simulink model "SensorlessFOC"  (R2026b)
settings: Solver=ode4  StopTime=experimentCfg.Duration  FixedStep=experimentCfg.Step
PostLoadFcn:
  | addpath(fullfile(fileparts(get_param(bdroot,'FileName')),'..','build_process'));initialize_sensorless_foc(bdroot);
model workspace (MAT data in the model file):
  currentCfg.Ts = 5e-05
  currentCfg.BandwidthHz = 500
  currentCfg.Kpd = 3.14159265359
  currentCfg.Kpq = 3.14159265359
  currentCfg.Kid = 1570.79632679
  currentCfg.Kiq = 1570.79632679
  currentCfg.Kaw = 20000
  deadtimeCfg.DeadTime = 2e-06
  deadtimeCfg.DeviceDrop = 0
  deadtimeCfg.CurrentBlend = 0.1
  deadtimeCfg.ModelEnable = 0
  deadtimeCfg.CompensationEnable = 0
  deadtimeCfg.CompensationScale = 1
  deadtimeCfg.SwitchingStep = 1e-07
  experimentCfg.UseInverter = 1
  experimentCfg.UseTiming = 1
  experimentCfg.Step = 5e-06
  experimentCfg.LogTs = 5e-05
  experimentCfg.Duration = 2
  focCfg.Direction = 1
  focCfg.SpeedReference = 80
  focCfg.SpeedInitial = 0
  focCfg.CommandTime = 0.05
  focCfg.LoadTorque = 0.1
  focCfg.LoadTime = 0.9
  focCfg.Enable = 1
  focCfg.Reset = 0
  focCfg.ObserverEnable = 1
  focCfg.CurrentMax = 8
  focCfg.Kt = 0.21
  focCfg.VoltageAlignmentEnable = 1
  focCfg.AlignmentVoltageGain = 0.5
  focCfg.FrameCorrectionTolerance = 1e-10
  handoverCfg.Ts = 5e-05
  handoverCfg.MinOmega = 100
  handoverCfg.MaxSpeedGap = 80
  handoverCfg.MaxPhaseGap = 0.9
  handoverCfg.MaxResidual = 1.5
  handoverCfg.CaptureTime = 0.01
  handoverCfg.BlendTime = 0.1
  handoverCfg.LossTime = 0.001
  handoverCfg.MaxPhaseInnovation = 0.15
  handoverCfg.AllowFlying = 0
  handoverCfg.Samples = [200; 2000; 20]
  handoverCfg.Vector = [5e-05; 100; 80; 0.9; 1.5; 200; 2000; 20; 0.15; 0]
  handoverCfg.State0 = [0; 0; 0; 0; 0; 0; 0; 0; 0]
  inverterCfg.Vdc = 48
  inverterCfg.MinDuty = 0.02
  inverterCfg.PwmTs = 5e-05
  inverterCfg.LinearLimit = 26.6043004043
  motionCfg.Ts = 0.001
  motionCfg.NaturalFrequency = 20
  motionCfg.Damping = 0.9
  motionCfg.Kt = 0.21
  motionCfg.Kp = 0.0852380952381
  motionCfg.Ki = 0.952380952381
  motionCfg.Kaw = 20
  motionCfg.PositionKp = 8
  motionCfg.SpeedLimit = 120
  motionCfg.AccelerationLimit = 200
  motionCfg.CurrentLimit = 8
  pllCfg.Ts = 5e-05
  pllCfg.NaturalFrequency = 40
  pllCfg.Damping = 0.707
  pllCfg.Kp = 355.376960974
  pllCfg.Ki = 63165.468167
  pllCfg.Kaw = 502.654824574
  pllCfg.OmegaMax = 1500
  pllCfg.MinMagnitude = 1
  pllCfg.LockError = 0.12
  pllCfg.LockSamples = 100
  pllCfg.Theta0 = 0
  pllCfg.Omega0 = 0
  pmsmCfg.Rs = 0.5
  pmsmCfg.Ld = 0.001
  pmsmCfg.Lq = 0.001
  pmsmCfg.Flux = 0.035
  pmsmCfg.PolePairs = 4
  pmsmCfg.J = 0.0005
  pmsmCfg.B = 0.0001
  pmsmCfg.Id0 = 0
  pmsmCfg.Iq0 = 0
  pmsmCfg.Speed0 = 0
  pmsmCfg.Position0 = 0.1
  refCfg.SpeedTs = 0.001
  refCfg.SpeedKp = 0.0179
  refCfg.SpeedKi = 0.2
  refCfg.SpeedKaw = 1000
  smoCfg.Ts = 5e-05
  smoCfg.Rs = 0.5
  smoCfg.L = 0.001
  smoCfg.Flux = 0.035
  smoCfg.PolePairs = 4
  smoCfg.SlidingGain = 30
  smoCfg.Boundary = 1
  smoCfg.FilterHz = 600
  smoCfg.MinEmf = 1
  smoCfg.MinOmega = 30
  smoCfg.Compensate = 1
  smoCfg.A = 0.975309912028
  smoCfg.B = 0.0493801759433
  smoCfg.FilterA = 0.828204181307
  smoCfg.BoundaryPole = -0.506095366272
  startupCfg.Ts = 5e-05
  startupCfg.Theta0 = 0
  startupCfg.AlignCurrent = 2
  startupCfg.StartupCurrent = 3
  startupCfg.FinalOmega = 250
  startupCfg.FlyingCaptureTime = 0.03
  startupCfg.PrealignTime = 0.06
  startupCfg.PrealignRampTime = 0.03
  startupCfg.AlignTime = 0.08
  startupCfg.AlignRampTime = 0.04
  startupCfg.OmegaRampTime = 0.35
  startupCfg.CurrentRampTime = 0.05
  startupCfg.MinCaptureOmega = 150
  startupCfg.MaxIFTime = 0.8
  startupCfg.Samples = [600 1200 600 1600 800 7000 1000 16000]
  startupCfg.Vector = [5e-05; 0; 2; 3; 250; 600; 1200; 600; 1600; 800; 7000; 1000; 16000; 150]
  startupCfg.State0 = [0; 0; 0; 0; 0]
  testStim.time = [0 5e-05 0.0001 0.00015 0.0002 0.00025 0.0003 0.00035 0.0004 0.00045 0.0005 0.00055 ... (40001 elements, 40001x1)]
  testStim.signals.values = [0 0 0 0 0 0 0 0 0 0 0 0 ... (240006 elements, 40001x6)]
  testStim.signals.dimensions = 6
  timingCfg.Ts = 5e-05
  timingCfg.FeedbackTicks = 0
  timingCfg.ActuationTicks = 1
libraries: ClarkePark x14, Inverter x3, CurrentControl x2, PMSMPlant x2, Deadtime x2, SensorlessHandover x1, CurrentReference x1, SensorlessStartup x1, SlidingModeObserver x1, ControlTiming x1
settings Model: Creator=24322  LastModifiedBy=24322

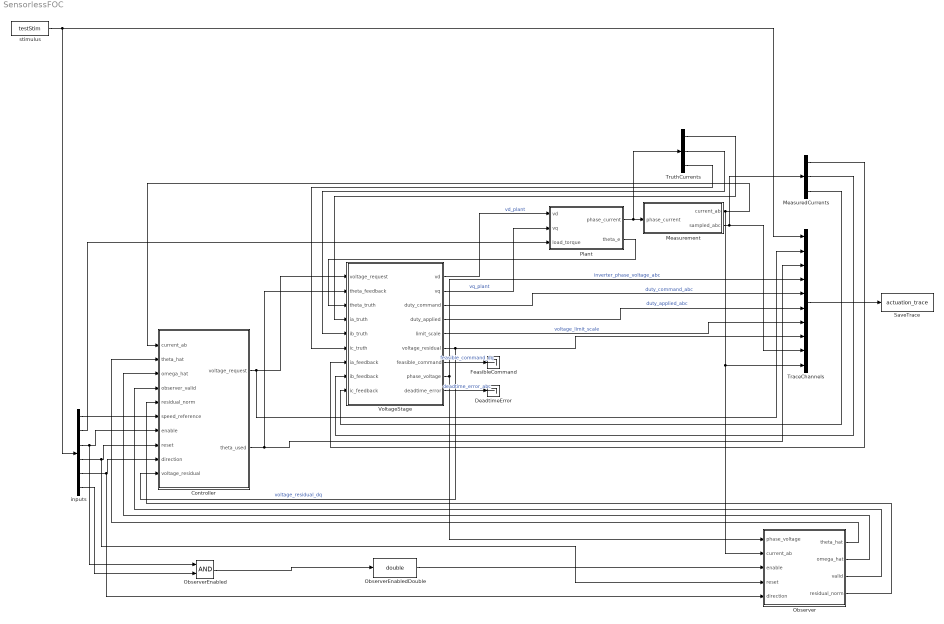
== system SensorlessFOC ==
  Controller : Subsystem
  DeadtimeError : Terminator
  FeasibleCommand : Terminator
  MeasuredCurrents : Demux  Outputs=3
  Measurement : Subsystem
  Observer : Subsystem
  ObserverEnabled : Logic  IconShape=distinctive  AllPortsSameDT=off  OutDataTypeStr=boolean
  ObserverEnabledDouble : DataTypeConversion  OutDataTypeStr=double  SaturateOnIntegerOverflow=off  RndMeth=Floor
  Plant : Subsystem
  SaveTrace : ToWorkspace  VariableName=actuation_trace  SaveFormat=Structure With Time  SampleTime=currentCfg.Ts
  TraceChannels : Mux  Inputs=10
  TruthCurrents : Demux  Outputs=3
  VoltageStage : Subsystem
  inputs : Demux  Outputs=6
  stimulus : FromWorkspace  VariableName=testStim  SampleTime=currentCfg.Ts  Interpolate=off  OutputAfterFinalValue=Holding final value
  wires:
  VoltageStage/5(limit_scale) -> TraceChannels/7  "voltage_limit_scale"
  VoltageStage/4(duty_applied) -> TraceChannels/6  "duty_applied_abc"
  VoltageStage/3(duty_command) -> TraceChannels/5  "duty_command_abc"
  TraceChannels/1 -> SaveTrace/1
  MeasuredCurrents/3 -> VoltageStage/9(ic_feedback)
  TruthCurrents/3 -> VoltageStage/6(ic_truth)
  MeasuredCurrents/2 -> VoltageStage/8(ib_feedback)
  TruthCurrents/2 -> VoltageStage/5(ib_truth)
  MeasuredCurrents/1 -> VoltageStage/7(ia_feedback)
  TruthCurrents/1 -> VoltageStage/4(ia_truth)
  VoltageStage/9(deadtime_error) -> DeadtimeError/1  "deadtime_error_abc"
  VoltageStage/7(feasible_command) -> FeasibleCommand/1  "feasible_command_dq"
  VoltageStage/6(voltage_residual) -> Controller/10(voltage_residual), TraceChannels/8  "voltage_residual_dq"
  inputs/1 -> Controller/6(speed_reference)
  Observer/4(residual_norm) -> Controller/5(residual_norm)
  Observer/3(valid) -> Controller/4(observer_valid)
  Observer/2(omega_hat) -> Controller/3(omega_hat)
  Observer/1(theta_hat) -> Controller/2(theta_hat)
  inputs/5 -> Observer/5(direction), Controller/9(direction)
  inputs/4 -> Observer/4(reset), Controller/8(reset)
  ObserverEnabledDouble/1 -> Observer/3(enable)
  Measurement/1(current_ab) -> TraceChannels/10, Observer/2(current_ab), Controller/1(current_ab)
  VoltageStage/8(phase_voltage) -> Observer/1(phase_voltage), TraceChannels/4  "inverter_phase_voltage_abc"
  Measurement/2(sampled_abc) -> MeasuredCurrents/1, TraceChannels/9
  Plant/1(phase_current) -> Measurement/1(phase_current), TruthCurrents/1
  inputs/2 -> Plant/3(load_torque)
  VoltageStage/2(vq) -> Plant/2(vq)  "vq_plant"
  VoltageStage/1(vd) -> Plant/1(vd)  "vd_plant"
  Plant/2(theta_e) -> VoltageStage/3(theta_truth)
  Controller/2(theta_used) -> VoltageStage/2(theta_feedback), TraceChannels/3
  Controller/1(voltage_request) -> VoltageStage/1(voltage_request), TraceChannels/2
  ObserverEnabled/1 -> ObserverEnabledDouble/1
  inputs/6 -> ObserverEnabled/2
  inputs/3 -> ObserverEnabled/1, Controller/7(enable)
  stimulus/1 -> inputs/1, TraceChannels/1

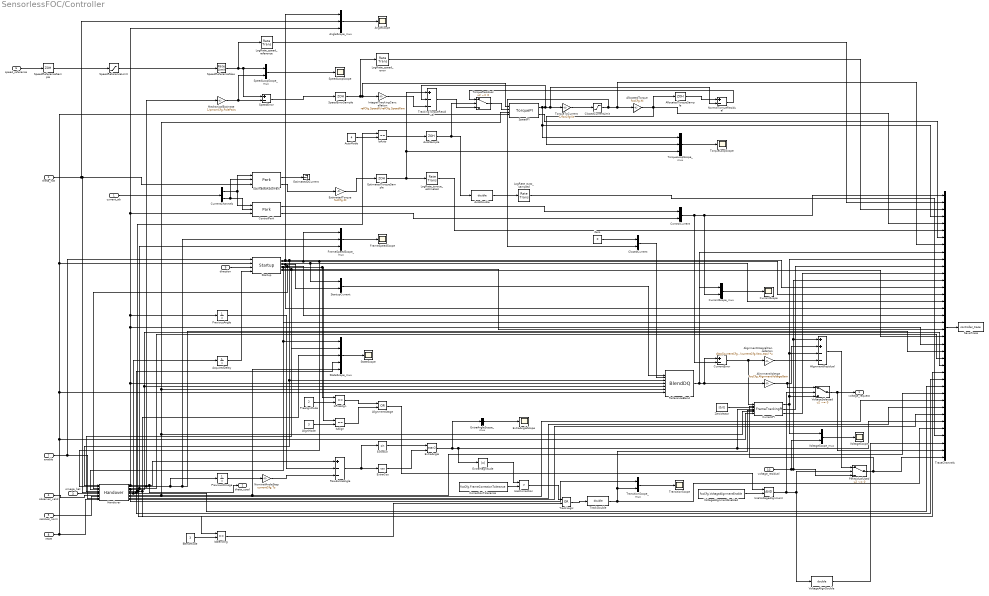
== system SensorlessFOC/Controller ==
  current_ab : Inport
  theta_hat : Inport  Port=2
  omega_hat : Inport  Port=3
  observer_valid : Inport  Port=4
  residual_norm : Inport  Port=5
  speed_reference : Inport  Port=6
  enable : Inport  Port=7
  reset : Inport  Port=8
  direction : Inport  Port=9
  voltage_residual : Inport  Port=10
  AcquiredDelay : UnitDelay  SampleTime=currentCfg.Ts
  AlignMode : Constant  Value=3
  AlignmentIntegralCancellation : Gain  Gain=diag([currentCfg.Kid,currentCfg.Kiq])/max(currentCfg.Kaw,eps)  Multiplication=Matrix(K*u)
  AlignmentResidual : Sum  Inputs=++--
  AlignmentStage : Logic  Operator=OR  IconShape=distinctive  AllPortsSameDT=off  OutDataTypeStr=boolean
  AlignmentVoltage : Gain  Gain=focCfg.AlignmentVoltageGain
  AllocatedTorque : Gain  Gain=focCfg.Kt
  AllocatedTorqueSample : ZeroOrderHold  SampleTime=refCfg.SpeedTs
  AngleScope : Scope
  AngleScope_mux : Mux  Inputs=3
  AutoDouble : DataTypeConversion  OutDataTypeStr=double  SaturateOnIntegerOverflow=off  RndMeth=Floor
  AutoMode : Constant  Value=4
  AutoSample : ZeroOrderHold  SampleTime=refCfg.SpeedTs
  BlendMode : Constant  Value=3
  ClosedCurrent : Mux  Inputs=2
  ClosedCurrentLimit : Saturate  UpperLimit=focCfg.CurrentMax  LowerLimit=-focCfg.CurrentMax
  ControlCurrent : Mux  Inputs=2
  ControlPark : ClarkePark/Park  SystemSampleTime=-1  VariantActivationTime=update diagram  EmptyChoice=off  PassThrough=off  PassThroughVariantControl=(default)  EmptyChoiceVariantControl=(default)  AllowFlexibleInterface=on  Latency=0  AutoFrameSizeCalculation=off
  CorrectionTolerance : Constant  Value=focCfg.FrameCorrectionTolerance
  CurrentChannels : Demux  Outputs=2
  CurrentError : Sum  Inputs=+-
  CurrentPI : CurrentControl/FrameTrackingPI  currentCfg=currentCfg
  CurrentScope : Scope
  CurrentScope_mux : Mux  Inputs=2
  EstimatedDCurrent : Terminator
  EstimatedRotorPark : ClarkePark/Park  SystemSampleTime=-1  VariantActivationTime=update diagram  EmptyChoice=off  PassThrough=off  PassThroughVariantControl=(default)  EmptyChoiceVariantControl=(default)  AllowFlexibleInterface=on  Latency=0  AutoFrameSizeCalculation=off
  EstimatedTorque : Gain  Gain=focCfg.Kt
  EstimatedTorqueSample : ZeroOrderHold  SampleTime=refCfg.SpeedTs
  ExtraAngle : Trigonometry  Operator=atan2
  ExtraAngleScope : Scope
  ExtraAngleScope_mux : Mux  Inputs=1
  ExtraCos : Trigonometry  Operator=cos
  ExtraMagnitude : Abs  SaturateOnIntegerOverflow=off
  ExtraSin : Trigonometry
  FrameSpeedScope : Scope
  FrameSpeedScope_mux : Mux  Inputs=3
  Handover : SensorlessHandover/Handover  handoverCfg=handoverCfg
  HasCorrection : RelationalOperator  Operator=>  OutDataTypeStr=boolean  RndMeth=Simplest  InputSameDT=off
  IntegralTrackingCancellation : Gain  Gain=refCfg.SpeedKi/refCfg.SpeedKaw
  IsAlign : RelationalOperator  Operator===  OutDataTypeStr=boolean  RndMeth=Simplest  InputSameDT=off
  IsAuto : RelationalOperator  Operator===  OutDataTypeStr=boolean  RndMeth=Simplest  InputSameDT=off
  IsBlending : RelationalOperator  Operator===  OutDataTypeStr=boolean  RndMeth=Simplest  InputSameDT=off
  IsPrealign : RelationalOperator  Operator===  OutDataTypeStr=boolean  RndMeth=Simplest  InputSameDT=off
  LogRate_auto_sampled : RateTransition  Integrity=off  Deterministic=off  OutPortSampleTime=currentCfg.Ts
  LogRate_speed_error : RateTransition  Integrity=off  Deterministic=off  OutPortSampleTime=currentCfg.Ts
  LogRate_speed_reference : RateTransition  Integrity=off  Deterministic=off  OutPortSampleTime=currentCfg.Ts
  LogRate_torque_estimated : RateTransition  Integrity=off  Deterministic=off  OutPortSampleTime=currentCfg.Ts
  MechanicalEstimate : Gain  Gain=1/pmsmCfg.PolePairs
  NominalAngleStep : Gain  Gain=currentCfg.Ts
  NormalTorqueResidual : Sum  Inputs=+-
  PIResidualUsed : Switch  Criteria=u2 ~= 0  SaturateOnIntegerOverflow=off  InputSameDT=off
  PrealignMode : Constant  Value=2
  PreviousAngle : UnitDelay  SampleTime=currentCfg.Ts
  PreviousOmega : UnitDelay  SampleTime=currentCfg.Ts
  RawExtraAngle : Sum  Inputs=+--
  ReferenceBlend : ClarkePark/BlendDQ  SystemSampleTime=-1  VariantActivationTime=update diagram  EmptyChoice=off  PassThrough=off  PassThroughVariantControl=(default)  EmptyChoiceVariantControl=(default)  AllowFlexibleInterface=on  Latency=0  AutoFrameSizeCalculation=off
  SaveTrace : ToWorkspace  VariableName=controller_trace  SaveFormat=Structure With Time  SampleTime=currentCfg.Ts
  SpeedError : Sum  Inputs=+-
  SpeedErrorSample : ZeroOrderHold  SampleTime=refCfg.SpeedTs
  SpeedLoopScope : Scope
  SpeedLoopScope_mux : Mux  Inputs=2
  SpeedPI : CurrentReference/TorquePI  SystemSampleTime=-1  VariantActivationTime=update diagram  EmptyChoice=off  PassThrough=off  PassThroughVariantControl=(default)  EmptyChoiceVariantControl=(default)  AllowFlexibleInterface=on  Latency=0  AutoFrameSizeCalculation=off
  SpeedReferenceLimit : Saturate  UpperLimit=motionCfg.SpeedLimit  LowerLimit=-motionCfg.SpeedLimit
  SpeedReferenceSample : ZeroOrderHold  SampleTime=refCfg.SpeedTs
  SpeedReferenceSlew : RateLimiter  RisingSlewLimit=motionCfg.AccelerationLimit  FallingSlewLimit=-motionCfg.AccelerationLimit  SampleTimeMode=inherited
  Startup : SensorlessStartup/Startup  startupCfg=startupCfg
  StartupCurrent : Mux  Inputs=2
  StateScope : Scope
  StateScope_mux : Mux  Inputs=5
  TorqueLoopScope : Scope
  TorqueLoopScope_mux : Mux  Inputs=3
  TorqueResidual : Switch  Criteria=u2 ~= 0  SaturateOnIntegerOverflow=off  InputSameDT=off
  TorqueToCurrent : Gain  Gain=1/focCfg.Kt
  TraceChannels : Mux  Inputs=38
  TrackDouble : DataTypeConversion  OutDataTypeStr=double  SaturateOnIntegerOverflow=off  RndMeth=Floor
  TrackLogic : Logic  Operator=OR  IconShape=distinctive  AllPortsSameDT=off  OutDataTypeStr=boolean
  TrackingTorqueResidual : Sum  Inputs=+--
  TransitionScope : Scope
  TransitionScope_mux : Mux  Inputs=2
  UseVoltageAlignment : Logic  IconShape=distinctive  AllPortsSameDT=off  OutDataTypeStr=boolean
  VoltageAlignDouble : DataTypeConversion  OutDataTypeStr=double  SaturateOnIntegerOverflow=off  RndMeth=Floor
  VoltageAlignmentEnabled : Constant  Value=focCfg.VoltageAlignmentEnable
  VoltageScope : Scope
  VoltageScope_mux : Mux  Inputs=2
  VoltageSelected : Switch  Criteria=u2 ~= 0  SaturateOnIntegerOverflow=off  InputSameDT=off
  Zero : Constant  Value=0
  ZeroVector : Constant  Value=[0;0]
  voltage_request : Outport
  theta_used : Outport  Port=2
  wires:
  VoltageAlignDouble/1 -> TraceChannels/36
  LogRate_auto_sampled/1 -> TraceChannels/35
  LogRate_torque_estimated/1 -> TraceChannels/6
  LogRate_speed_error/1 -> TraceChannels/3
  LogRate_speed_reference/1 -> TraceChannels/2
  VoltageSelected/1 -> voltage_request/1, TraceChannels/37
  PIResidualUsed/1 -> CurrentPI/2, TraceChannels/38
  AlignmentResidual/1 -> PIResidualUsed/1
  AlignmentIntegralCancellation/1 -> AlignmentResidual/4
  AlignmentVoltage/1 -> AlignmentResidual/2, VoltageSelected/1
  UseVoltageAlignment/1 -> VoltageAlignDouble/1, PIResidualUsed/2, VoltageSelected/2
  VoltageAlignmentEnabled/1 -> UseVoltageAlignment/2
  AlignmentStage/1 -> UseVoltageAlignment/1
  IsAlign/1 -> AlignmentStage/2
  IsPrealign/1 -> AlignmentStage/1
  AlignMode/1 -> IsAlign/2
  PrealignMode/1 -> IsPrealign/2
  current_ab/1 -> CurrentChannels/1
  CurrentChannels/1 -> EstimatedRotorPark/1, ControlPark/1
  CurrentChannels/2 -> EstimatedRotorPark/2, ControlPark/2
  Handover/1 -> RawExtraAngle/1, theta_used/1, ControlPark/3, AngleScope_mux/3, PreviousAngle/1, TraceChannels/22, ReferenceBlend/4
  ControlPark/1 -> ControlCurrent/1
  ControlPark/2 -> ControlCurrent/2
  theta_hat/1 -> EstimatedRotorPark/3, Handover/6, AngleScope_mux/2
  EstimatedRotorPark/1 -> EstimatedDCurrent/1
  EstimatedRotorPark/2 -> EstimatedTorque/1
  EstimatedTorque/1 -> EstimatedTorqueSample/1
  enable/1 -> Handover/10, Startup/1
  reset/1 -> SpeedPI/4, Startup/2, ReferenceBlend/7, CurrentPI/7, Handover/11
  direction/1 -> Startup/3
  AcquiredDelay/1 -> Startup/4
  Handover/7 -> AcquiredDelay/1, TraceChannels/28
  Startup/1 -> Handover/1, ReferenceBlend/3, TraceChannels/14, AngleScope_mux/1
  Startup/2 -> TraceChannels/15, Handover/2, FrameSpeedScope_mux/1
  Startup/5 -> TraceChannels/18, Handover/3
  Startup/6 -> StateScope_mux/1, Handover/4, IsPrealign/1, IsAlign/1, TraceChannels/19
  Startup/7 -> TraceChannels/20, Handover/5, StateScope_mux/2
  omega_hat/1 -> Handover/7
  observer_valid/1 -> Handover/8
  residual_norm/1 -> Handover/9
  speed_reference/1 -> SpeedReferenceSample/1
  SpeedReferenceSample/1 -> SpeedReferenceLimit/1
  SpeedReferenceLimit/1 -> SpeedReferenceSlew/1
  SpeedReferenceSlew/1 -> SpeedError/1, SpeedLoopScope_mux/1, LogRate_speed_reference/1
  MechanicalEstimate/1 -> SpeedLoopScope_mux/2, SpeedError/2
  SpeedError/1 -> SpeedErrorSample/1
  SpeedErrorSample/1 -> SpeedPI/1, IntegralTrackingCancellation/1, LogRate_speed_error/1
  TorqueResidual/1 -> SpeedPI/2
  Handover/8 -> StateScope_mux/5, TraceChannels/29, ReferenceBlend/6, SpeedPI/3, CurrentPI/6
  SpeedPI/1 -> TraceChannels/4, TorqueLoopScope_mux/1, TorqueToCurrent/1, NormalTorqueResidual/2, TrackingTorqueResidual/2
  TorqueToCurrent/1 -> ClosedCurrentLimit/1
  ClosedCurrentLimit/1 -> AllocatedTorque/1, TraceChannels/8, ClosedCurrent/2
  AllocatedTorque/1 -> AllocatedTorqueSample/1, TraceChannels/5, TorqueLoopScope_mux/2
  AllocatedTorqueSample/1 -> NormalTorqueResidual/1
  EstimatedTorqueSample/1 -> TorqueLoopScope_mux/3, TrackingTorqueResidual/1, LogRate_torque_estimated/1
  IntegralTrackingCancellation/1 -> TrackingTorqueResidual/3
  Handover/5 -> StateScope_mux/3, TraceChannels/26, IsBlending/1, IsAuto/1
  AutoMode/1 -> IsAuto/2
  IsAuto/1 -> AutoSample/1
  AutoSample/1 -> TorqueResidual/2, AutoDouble/1
  NormalTorqueResidual/1 -> TorqueResidual/1
  TrackingTorqueResidual/1 -> TorqueResidual/3
  Startup/3 -> TraceChannels/16, StartupCurrent/1
  Startup/4 -> TraceChannels/17, StartupCurrent/2
  Zero/1 -> ClosedCurrent/1
  StartupCurrent/1 -> ReferenceBlend/1
  ClosedCurrent/1 -> ReferenceBlend/2
  Handover/4 -> ReferenceBlend/5, TraceChannels/25, TransitionScope_mux/1
  ReferenceBlend/1 -> CurrentError/1, AlignmentVoltage/1, TraceChannels/9, CurrentScope_mux/1
  ControlCurrent/1 -> CurrentScope_mux/2, TraceChannels/1, CurrentError/2
  CurrentError/1 -> CurrentPI/1, AlignmentIntegralCancellation/1
  voltage_residual/1 -> TraceChannels/13, AlignmentResidual/1, PIResidualUsed/3, VoltageScope_mux/2
  ZeroVector/1 -> CurrentPI/3
  ExtraAngle/1 -> CurrentPI/4, TraceChannels/33, ExtraMagnitude/1, ExtraAngleScope_mux/1
  TrackDouble/1 -> CurrentPI/5, TransitionScope_mux/2, TraceChannels/34
  CurrentPI/1 -> TraceChannels/10, AlignmentResidual/3, VoltageSelected/3, VoltageScope_mux/1
  Handover/2 -> FrameSpeedScope_mux/2, TraceChannels/23, PreviousOmega/1, MechanicalEstimate/1
  PreviousOmega/1 -> NominalAngleStep/1
  PreviousAngle/1 -> RawExtraAngle/2
  NominalAngleStep/1 -> RawExtraAngle/3
  RawExtraAngle/1 -> ExtraCos/1, ExtraSin/1
  ExtraSin/1 -> ExtraAngle/1
  ExtraCos/1 -> ExtraAngle/2
  ExtraMagnitude/1 -> HasCorrection/1
  CorrectionTolerance/1 -> HasCorrection/2
  BlendMode/1 -> IsBlending/2
  HasCorrection/1 -> TrackLogic/1
  IsBlending/1 -> TrackLogic/2
  TrackLogic/1 -> TrackDouble/1
  TraceChannels/1 -> SaveTrace/1
  SpeedPI/2 -> TraceChannels/7
  CurrentPI/2 -> TraceChannels/11
  CurrentPI/3 -> TraceChannels/12
  Startup/8 -> TraceChannels/21
  Handover/3 -> FrameSpeedScope_mux/3, TraceChannels/24
  Handover/6 -> StateScope_mux/4, TraceChannels/27
  Handover/9 -> TraceChannels/30
  Handover/10 -> TraceChannels/31
  Handover/11 -> TraceChannels/32
  AutoDouble/1 -> LogRate_auto_sampled/1
  CurrentScope_mux/1 -> CurrentScope/1
  AngleScope_mux/1 -> AngleScope/1
  FrameSpeedScope_mux/1 -> FrameSpeedScope/1
  TransitionScope_mux/1 -> TransitionScope/1
  ExtraAngleScope_mux/1 -> ExtraAngleScope/1
  StateScope_mux/1 -> StateScope/1
  SpeedLoopScope_mux/1 -> SpeedLoopScope/1
  TorqueLoopScope_mux/1 -> TorqueLoopScope/1
  VoltageScope_mux/1 -> VoltageScope/1

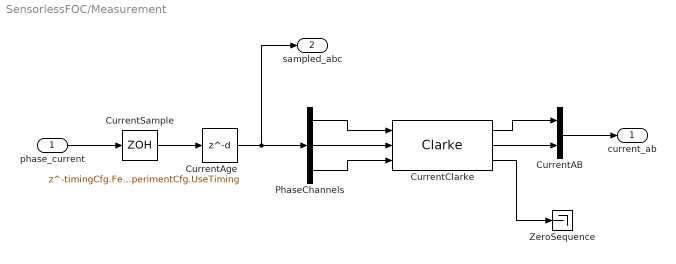
== system SensorlessFOC/Measurement ==
  phase_current : Inport
  CurrentAB : Mux  Inputs=2
  CurrentAge : Delay  DelayLength=timingCfg.FeedbackTicks*experimentCfg.UseTiming  InitialCondition=0  SampleTime=timingCfg.Ts
  CurrentClarke : ClarkePark/Clarke  SystemSampleTime=-1  VariantActivationTime=update diagram  EmptyChoice=off  PassThrough=off  PassThroughVariantControl=(default)  EmptyChoiceVariantControl=(default)  AllowFlexibleInterface=on  Latency=0  AutoFrameSizeCalculation=off
  CurrentSample : ZeroOrderHold  SampleTime=timingCfg.Ts
  PhaseChannels : Demux  Outputs=3
  ZeroSequence : Terminator
  current_ab : Outport
  sampled_abc : Outport  Port=2
  wires:
  PhaseChannels/3 -> CurrentClarke/3
  PhaseChannels/2 -> CurrentClarke/2
  PhaseChannels/1 -> CurrentClarke/1
  CurrentAB/1 -> current_ab/1
  CurrentClarke/3 -> ZeroSequence/1
  CurrentClarke/2 -> CurrentAB/2
  CurrentClarke/1 -> CurrentAB/1
  CurrentAge/1 -> PhaseChannels/1, sampled_abc/1
  CurrentSample/1 -> CurrentAge/1
  phase_current/1 -> CurrentSample/1

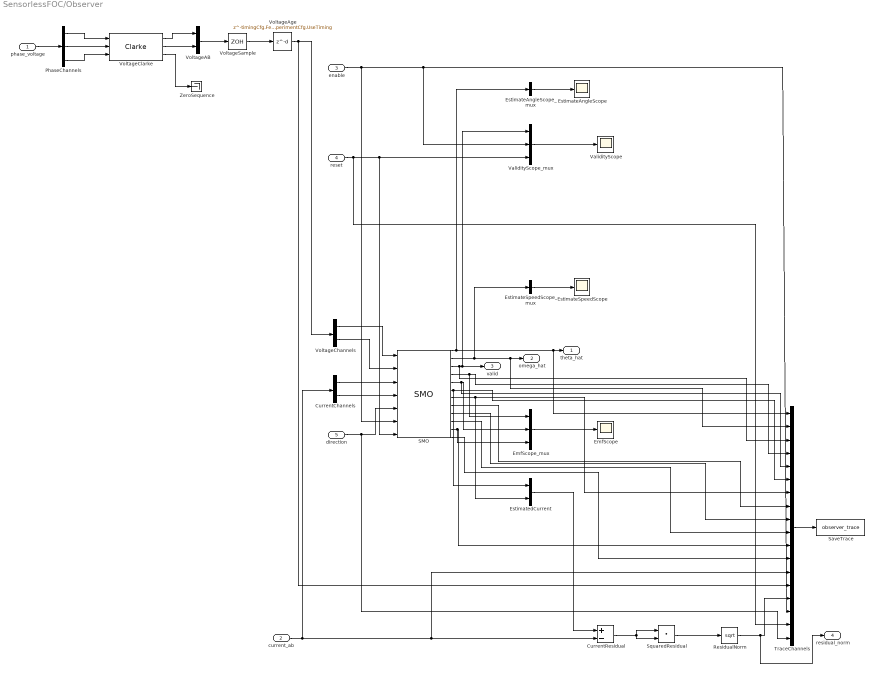
== system SensorlessFOC/Observer ==
  phase_voltage : Inport
  current_ab : Inport  Port=2
  enable : Inport  Port=3
  reset : Inport  Port=4
  direction : Inport  Port=5
  CurrentChannels : Demux  Outputs=2
  CurrentResidual : Sum  Inputs=+-
  EmfScope : Scope
  EmfScope_mux : Mux  Inputs=3
  EstimateAngleScope : Scope
  EstimateAngleScope_mux : Mux  Inputs=1
  EstimateSpeedScope : Scope
  EstimateSpeedScope_mux : Mux  Inputs=1
  EstimatedCurrent : Mux  Inputs=2
  PhaseChannels : Demux  Outputs=3
  ResidualNorm : Sqrt
  SMO : SlidingModeObserver/SMO  SystemSampleTime=-1  VariantActivationTime=update diagram  EmptyChoice=off  PassThrough=off  PassThroughVariantControl=(default)  EmptyChoiceVariantControl=(default)  AllowFlexibleInterface=on  Latency=0  AutoFrameSizeCalculation=off
  SaveTrace : ToWorkspace  VariableName=observer_trace  SaveFormat=Structure With Time  SampleTime=currentCfg.Ts
  SquaredResidual : DotProduct  OutDataTypeStr=Inherit: Inherit via internal rule
  TraceChannels : Mux  Inputs=18
  ValidityScope : Scope
  ValidityScope_mux : Mux  Inputs=3
  VoltageAB : Mux  Inputs=2
  VoltageAge : Delay  DelayLength=timingCfg.FeedbackTicks*experimentCfg.UseTiming  InitialCondition=0  SampleTime=timingCfg.Ts
  VoltageChannels : Demux  Outputs=2
  VoltageClarke : ClarkePark/Clarke  SystemSampleTime=-1  VariantActivationTime=update diagram  EmptyChoice=off  PassThrough=off  PassThroughVariantControl=(default)  EmptyChoiceVariantControl=(default)  AllowFlexibleInterface=on  Latency=0  AutoFrameSizeCalculation=off
  VoltageSample : ZeroOrderHold  SampleTime=timingCfg.Ts
  ZeroSequence : Terminator
  theta_hat : Outport
  omega_hat : Outport  Port=2
  valid : Outport  Port=3
  residual_norm : Outport  Port=4
  wires:
  ValidityScope_mux/1 -> ValidityScope/1
  EmfScope_mux/1 -> EmfScope/1
  EstimateSpeedScope_mux/1 -> EstimateSpeedScope/1
  EstimateAngleScope_mux/1 -> EstimateAngleScope/1
  SMO/12 -> TraceChannels/12
  SMO/11 -> TraceChannels/11, EmfScope_mux/3
  SMO/10 -> TraceChannels/10
  SMO/9 -> TraceChannels/9
  SMO/8 -> TraceChannels/8
  SMO/5 -> TraceChannels/5, EmfScope_mux/2
  SMO/4 -> TraceChannels/4, EmfScope_mux/1
  TraceChannels/1 -> SaveTrace/1
  PhaseChannels/3 -> VoltageClarke/3
  PhaseChannels/2 -> VoltageClarke/2
  PhaseChannels/1 -> VoltageClarke/1
  ResidualNorm/1 -> residual_norm/1, TraceChannels/15
  SquaredResidual/1 -> ResidualNorm/1
  CurrentResidual/1 -> SquaredResidual/1, SquaredResidual/2
  EstimatedCurrent/1 -> CurrentResidual/1
  SMO/7 -> EstimatedCurrent/2, TraceChannels/7
  SMO/6 -> EstimatedCurrent/1, TraceChannels/6
  SMO/3 -> valid/1, ValidityScope_mux/1, TraceChannels/3
  SMO/2 -> omega_hat/1, TraceChannels/2, EstimateSpeedScope_mux/1
  SMO/1 -> TraceChannels/1, theta_hat/1, EstimateAngleScope_mux/1
  reset/1 -> SMO/7, ValidityScope_mux/3, TraceChannels/17
  enable/1 -> ValidityScope_mux/2, TraceChannels/16, SMO/6
  direction/1 -> SMO/5, TraceChannels/18
  CurrentChannels/2 -> SMO/4
  CurrentChannels/1 -> SMO/3
  VoltageChannels/2 -> SMO/2
  VoltageChannels/1 -> SMO/1
  VoltageAge/1 -> VoltageChannels/1, TraceChannels/14
  VoltageSample/1 -> VoltageAge/1
  VoltageAB/1 -> VoltageSample/1
  VoltageClarke/3 -> ZeroSequence/1
  VoltageClarke/2 -> VoltageAB/2
  VoltageClarke/1 -> VoltageAB/1
  current_ab/1 -> CurrentResidual/2, TraceChannels/13, CurrentChannels/1
  phase_voltage/1 -> PhaseChannels/1

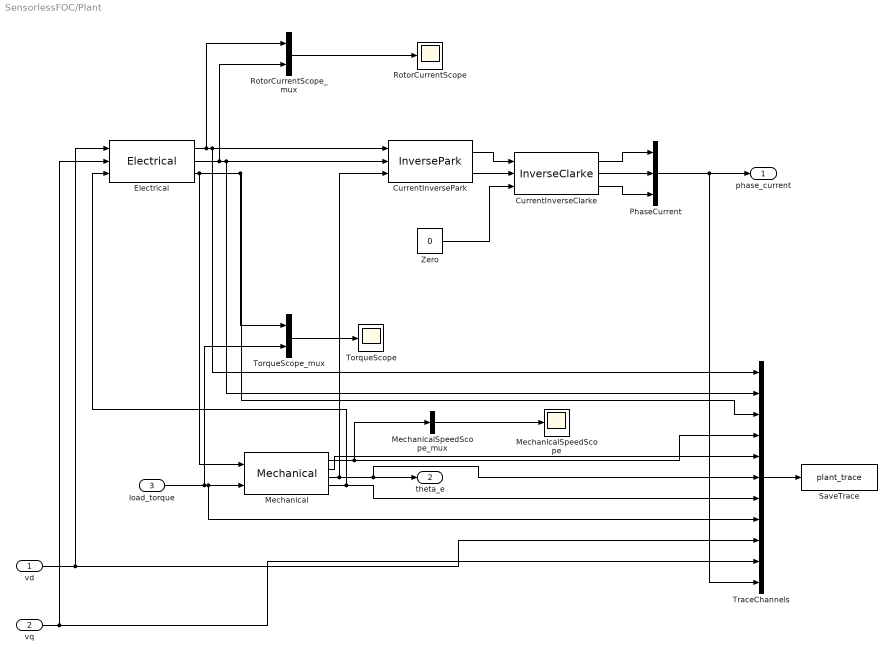
== system SensorlessFOC/Plant ==
  vd : Inport
  vq : Inport  Port=2
  load_torque : Inport  Port=3
  CurrentInverseClarke : ClarkePark/InverseClarke  SystemSampleTime=-1  VariantActivationTime=update diagram  EmptyChoice=off  PassThrough=off  PassThroughVariantControl=(default)  EmptyChoiceVariantControl=(default)  AllowFlexibleInterface=on  Latency=0  AutoFrameSizeCalculation=off
  CurrentInversePark : ClarkePark/InversePark  SystemSampleTime=-1  VariantActivationTime=update diagram  EmptyChoice=off  PassThrough=off  PassThroughVariantControl=(default)  EmptyChoiceVariantControl=(default)  AllowFlexibleInterface=on  Latency=0  AutoFrameSizeCalculation=off
  Electrical : PMSMPlant/Electrical  SystemSampleTime=-1  VariantActivationTime=update diagram  EmptyChoice=off  PassThrough=off  PassThroughVariantControl=(default)  EmptyChoiceVariantControl=(default)  AllowFlexibleInterface=on  Latency=0  AutoFrameSizeCalculation=off
  Mechanical : PMSMPlant/Mechanical  SystemSampleTime=-1  VariantActivationTime=update diagram  EmptyChoice=off  PassThrough=off  PassThroughVariantControl=(default)  EmptyChoiceVariantControl=(default)  AllowFlexibleInterface=on  Latency=0  AutoFrameSizeCalculation=off
  MechanicalSpeedScope : Scope
  MechanicalSpeedScope_mux : Mux  Inputs=1
  PhaseCurrent : Mux  Inputs=3
  RotorCurrentScope : Scope
  RotorCurrentScope_mux : Mux  Inputs=2
  SaveTrace : ToWorkspace  VariableName=plant_trace  SaveFormat=Structure With Time  SampleTime=currentCfg.Ts
  TorqueScope : Scope
  TorqueScope_mux : Mux  Inputs=2
  TraceChannels : Mux  Inputs=11
  Zero : Constant  Value=0
  phase_current : Outport
  theta_e : Outport  Port=2
  wires:
  TorqueScope_mux/1 -> TorqueScope/1
  MechanicalSpeedScope_mux/1 -> MechanicalSpeedScope/1
  RotorCurrentScope_mux/1 -> RotorCurrentScope/1
  Mechanical/2 -> TraceChannels/5
  Mechanical/1 -> TraceChannels/4, MechanicalSpeedScope_mux/1
  TraceChannels/1 -> SaveTrace/1
  CurrentInverseClarke/3 -> PhaseCurrent/3
  CurrentInverseClarke/2 -> PhaseCurrent/2
  CurrentInverseClarke/1 -> PhaseCurrent/1
  PhaseCurrent/1 -> TraceChannels/11, phase_current/1
  Zero/1 -> CurrentInverseClarke/3
  CurrentInversePark/2 -> CurrentInverseClarke/2
  CurrentInversePark/1 -> CurrentInverseClarke/1
  Mechanical/3 -> theta_e/1, TraceChannels/6, CurrentInversePark/3
  Electrical/2 -> CurrentInversePark/2, TraceChannels/2, RotorCurrentScope_mux/2
  Electrical/1 -> CurrentInversePark/1, TraceChannels/1, RotorCurrentScope_mux/1
  load_torque/1 -> Mechanical/2, TraceChannels/8, TorqueScope_mux/2
  Electrical/3 -> TraceChannels/3, TorqueScope_mux/1, Mechanical/1
  Mechanical/4 -> Electrical/3, TraceChannels/7
  vq/1 -> Electrical/2, TraceChannels/10
  vd/1 -> Electrical/1, TraceChannels/9

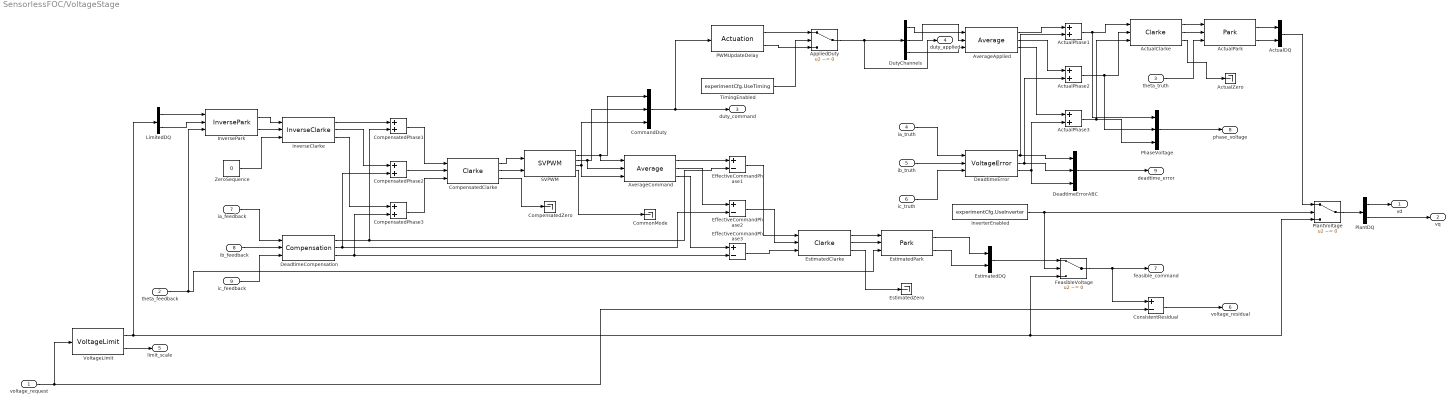
== system SensorlessFOC/VoltageStage ==
  voltage_request : Inport
  theta_feedback : Inport  Port=2
  theta_truth : Inport  Port=3
  ia_truth : Inport  Port=4
  ib_truth : Inport  Port=5
  ic_truth : Inport  Port=6
  ia_feedback : Inport  Port=7
  ib_feedback : Inport  Port=8
  ic_feedback : Inport  Port=9
  ActualClarke : ClarkePark/Clarke  SystemSampleTime=-1  VariantActivationTime=update diagram  EmptyChoice=off  PassThrough=off  PassThroughVariantControl=(default)  EmptyChoiceVariantControl=(default)  AllowFlexibleInterface=on  Latency=0  AutoFrameSizeCalculation=off
  ActualDQ : Mux  Inputs=2
  ActualPark : ClarkePark/Park  SystemSampleTime=-1  VariantActivationTime=update diagram  EmptyChoice=off  PassThrough=off  PassThroughVariantControl=(default)  EmptyChoiceVariantControl=(default)  AllowFlexibleInterface=on  Latency=0  AutoFrameSizeCalculation=off
  ActualPhase1 : Sum
  ActualPhase2 : Sum
  ActualPhase3 : Sum
  ActualZero : Terminator
  AppliedDuty : Switch  Criteria=u2 ~= 0  SaturateOnIntegerOverflow=off  InputSameDT=off
  AverageApplied : Inverter/Average  SystemSampleTime=-1  VariantActivationTime=update diagram  EmptyChoice=off  PassThrough=off  PassThroughVariantControl=(default)  EmptyChoiceVariantControl=(default)  AllowFlexibleInterface=on  Latency=0  AutoFrameSizeCalculation=off
  AverageCommand : Inverter/Average  SystemSampleTime=-1  VariantActivationTime=update diagram  EmptyChoice=off  PassThrough=off  PassThroughVariantControl=(default)  EmptyChoiceVariantControl=(default)  AllowFlexibleInterface=on  Latency=0  AutoFrameSizeCalculation=off
  CommandDuty : Mux  Inputs=3
  CommonMode : Terminator
  CompensatedClarke : ClarkePark/Clarke  SystemSampleTime=-1  VariantActivationTime=update diagram  EmptyChoice=off  PassThrough=off  PassThroughVariantControl=(default)  EmptyChoiceVariantControl=(default)  AllowFlexibleInterface=on  Latency=0  AutoFrameSizeCalculation=off
  CompensatedPhase1 : Sum
  CompensatedPhase2 : Sum
  CompensatedPhase3 : Sum
  CompensatedZero : Terminator
  ConsistentResidual : Sum  Inputs=+-
  DeadtimeCompensation : Deadtime/Compensation  SystemSampleTime=-1  VariantActivationTime=update diagram  EmptyChoice=off  PassThrough=off  PassThroughVariantControl=(default)  EmptyChoiceVariantControl=(default)  AllowFlexibleInterface=on  Latency=0  AutoFrameSizeCalculation=off
  DeadtimeError : Deadtime/VoltageError  SystemSampleTime=-1  VariantActivationTime=update diagram  EmptyChoice=off  PassThrough=off  PassThroughVariantControl=(default)  EmptyChoiceVariantControl=(default)  AllowFlexibleInterface=on  Latency=0  AutoFrameSizeCalculation=off
  DeadtimeErrorABC : Mux  Inputs=3
  DutyChannels : Demux  Outputs=3
  EffectiveCommandPhase1 : Sum  Inputs=+-
  EffectiveCommandPhase2 : Sum  Inputs=+-
  EffectiveCommandPhase3 : Sum  Inputs=+-
  EstimatedClarke : ClarkePark/Clarke  SystemSampleTime=-1  VariantActivationTime=update diagram  EmptyChoice=off  PassThrough=off  PassThroughVariantControl=(default)  EmptyChoiceVariantControl=(default)  AllowFlexibleInterface=on  Latency=0  AutoFrameSizeCalculation=off
  EstimatedDQ : Mux  Inputs=2
  EstimatedPark : ClarkePark/Park  SystemSampleTime=-1  VariantActivationTime=update diagram  EmptyChoice=off  PassThrough=off  PassThroughVariantControl=(default)  EmptyChoiceVariantControl=(default)  AllowFlexibleInterface=on  Latency=0  AutoFrameSizeCalculation=off
  EstimatedZero : Terminator
  FeasibleVoltage : Switch  Criteria=u2 ~= 0  SaturateOnIntegerOverflow=off  InputSameDT=off
  InverseClarke : ClarkePark/InverseClarke  SystemSampleTime=-1  VariantActivationTime=update diagram  EmptyChoice=off  PassThrough=off  PassThroughVariantControl=(default)  EmptyChoiceVariantControl=(default)  AllowFlexibleInterface=on  Latency=0  AutoFrameSizeCalculation=off
  InversePark : ClarkePark/InversePark  SystemSampleTime=-1  VariantActivationTime=update diagram  EmptyChoice=off  PassThrough=off  PassThroughVariantControl=(default)  EmptyChoiceVariantControl=(default)  AllowFlexibleInterface=on  Latency=0  AutoFrameSizeCalculation=off
  InverterEnabled : Constant  Value=experimentCfg.UseInverter
  LimitedDQ : Demux  Outputs=2
  PWMUpdateDelay : ControlTiming/Actuation  SystemSampleTime=-1  VariantActivationTime=update diagram  EmptyChoice=off  PassThrough=off  PassThroughVariantControl=(default)  EmptyChoiceVariantControl=(default)  AllowFlexibleInterface=on  Latency=0  AutoFrameSizeCalculation=off
  PhaseVoltage : Mux  Inputs=3
  PlantDQ : Demux  Outputs=2
  PlantVoltage : Switch  Criteria=u2 ~= 0  SaturateOnIntegerOverflow=off  InputSameDT=off
  SVPWM : Inverter/SVPWM  SystemSampleTime=-1  VariantActivationTime=update diagram  EmptyChoice=off  PassThrough=off  PassThroughVariantControl=(default)  EmptyChoiceVariantControl=(default)  AllowFlexibleInterface=on  Latency=0  AutoFrameSizeCalculation=off
  TimingEnabled : Constant  Value=experimentCfg.UseTiming
  VoltageLimit : CurrentControl/VoltageLimit  SystemSampleTime=-1  VariantActivationTime=update diagram  EmptyChoice=off  PassThrough=off  PassThroughVariantControl=(default)  EmptyChoiceVariantControl=(default)  AllowFlexibleInterface=on  Latency=0  AutoFrameSizeCalculation=off
  ZeroSequence : Constant  Value=0
  vd : Outport
  vq : Outport  Port=2
  duty_command : Outport  Port=3
  duty_applied : Outport  Port=4
  limit_scale : Outport  Port=5
  voltage_residual : Outport  Port=6
  feasible_command : Outport  Port=7
  phase_voltage : Outport  Port=8
  deadtime_error : Outport  Port=9
  wires:
  voltage_request/1 -> VoltageLimit/1, ConsistentResidual/2
  VoltageLimit/1 -> LimitedDQ/1, FeasibleVoltage/3, PlantVoltage/3
  LimitedDQ/1 -> InversePark/1
  LimitedDQ/2 -> InversePark/2
  theta_feedback/1 -> EstimatedPark/3, InversePark/3
  InversePark/1 -> InverseClarke/1
  InversePark/2 -> InverseClarke/2
  ZeroSequence/1 -> InverseClarke/3
  CompensatedClarke/1 -> SVPWM/1
  CompensatedClarke/2 -> SVPWM/2
  CompensatedClarke/3 -> CompensatedZero/1
  SVPWM/4 -> CommonMode/1
  CommandDuty/1 -> duty_command/1, PWMUpdateDelay/1
  PWMUpdateDelay/1 -> AppliedDuty/1
  TimingEnabled/1 -> AppliedDuty/2
  PWMUpdateDelay/2 -> AppliedDuty/3
  AppliedDuty/1 -> duty_applied/1, DutyChannels/1
  ActualClarke/1 -> ActualPark/1
  ActualClarke/2 -> ActualPark/2
  theta_truth/1 -> ActualPark/3
  ActualClarke/3 -> ActualZero/1
  EstimatedClarke/1 -> EstimatedPark/1
  EstimatedClarke/2 -> EstimatedPark/2
  EstimatedClarke/3 -> EstimatedZero/1
  ActualPark/1 -> ActualDQ/1
  ActualPark/2 -> ActualDQ/2
  EstimatedPark/1 -> EstimatedDQ/1
  EstimatedPark/2 -> EstimatedDQ/2
  ActualDQ/1 -> PlantVoltage/1
  InverterEnabled/1 -> FeasibleVoltage/2, PlantVoltage/2
  EstimatedDQ/1 -> FeasibleVoltage/1
  FeasibleVoltage/1 -> feasible_command/1, ConsistentResidual/1
  PlantVoltage/1 -> PlantDQ/1
  PlantDQ/1 -> vd/1
  PlantDQ/2 -> vq/1
  VoltageLimit/2 -> limit_scale/1
  ConsistentResidual/1 -> voltage_residual/1
  PhaseVoltage/1 -> phase_voltage/1
  DeadtimeErrorABC/1 -> deadtime_error/1
  ia_feedback/1 -> DeadtimeCompensation/1
  ia_truth/1 -> DeadtimeError/1
  InverseClarke/1 -> CompensatedPhase1/1
  DeadtimeCompensation/1 -> EffectiveCommandPhase1/2, CompensatedPhase1/2
  CompensatedPhase1/1 -> CompensatedClarke/1
  SVPWM/1 -> AverageCommand/1, CommandDuty/1
  DutyChannels/1 -> AverageApplied/1
  AverageApplied/1 -> ActualPhase1/1
  DeadtimeError/1 -> DeadtimeErrorABC/1, ActualPhase1/2
  ActualPhase1/1 -> PhaseVoltage/1, ActualClarke/1
  AverageCommand/1 -> EffectiveCommandPhase1/1
  EffectiveCommandPhase1/1 -> EstimatedClarke/1
  ib_feedback/1 -> DeadtimeCompensation/2
  ib_truth/1 -> DeadtimeError/2
  InverseClarke/2 -> CompensatedPhase2/1
  DeadtimeCompensation/2 -> EffectiveCommandPhase2/2, CompensatedPhase2/2
  CompensatedPhase2/1 -> CompensatedClarke/2
  SVPWM/2 -> AverageCommand/2, CommandDuty/2
  DutyChannels/2 -> AverageApplied/2
  AverageApplied/2 -> ActualPhase2/1
  DeadtimeError/2 -> DeadtimeErrorABC/2, ActualPhase2/2
  ActualPhase2/1 -> PhaseVoltage/2, ActualClarke/2
  AverageCommand/2 -> EffectiveCommandPhase2/1
  EffectiveCommandPhase2/1 -> EstimatedClarke/2
  ic_feedback/1 -> DeadtimeCompensation/3
  ic_truth/1 -> DeadtimeError/3
  InverseClarke/3 -> CompensatedPhase3/1
  DeadtimeCompensation/3 -> EffectiveCommandPhase3/2, CompensatedPhase3/2
  CompensatedPhase3/1 -> CompensatedClarke/3
  SVPWM/3 -> AverageCommand/3, CommandDuty/3
  DutyChannels/3 -> AverageApplied/3
  AverageApplied/3 -> ActualPhase3/1
  DeadtimeError/3 -> DeadtimeErrorABC/3, ActualPhase3/2
  ActualPhase3/1 -> PhaseVoltage/3, ActualClarke/3
  AverageCommand/3 -> EffectiveCommandPhase3/1
  EffectiveCommandPhase3/1 -> EstimatedClarke/3
